simulink model "Rail_RegenerativeBraking_TianjinMetro_MotorSelection_v1"  (R2025a)
settings: Solver=ode23tb  StartTime=0.0  StopTime=SCv1.scenario.stop_time  FixedStep=Ts  MaxStep=Ts  RelTol=1e-4  EnableMultiTasking=on
PreLoadFcn:
  | SCv1_root=fileparts(fileparts(get_param(bdroot,'FileName'))); run(fullfile(SCv1_root,'config','SC_v1_parameters.m')); clear SCv1_root;
model workspace (MAT data in the model file):
  MotorCandidateIDs : object (value not decoded)
  MotorSurrogateStatement = 'parameterized surrogate traction motor model based on published nameplate data'
  TianjinMetroBaseline : object (value not decoded)
undefined symbols (not defined in the file): DiscIntNeverNeededParam, flux, Ld, Lq, Pn, SCv1, Ts
libraries: spsSeriesRLCBranchLib x5, spsControlledCurrentSourceLib x3, spsCurrentMeasurementLib x3, spsVoltageMeasurementLib x3, powerlib_extras x2, spsDCVoltageSourceLib x1, spsDiodeLib x1, spsPermanentMagnetSynchronousMachineLib x1, simulink x1, spsUniversalBridgeLib x1, sps_lib x1
(part 2 of 2)

== matlab function Rail_RegenerativeBraking_TianjinMetro_MotorSelection_v1/VehicleDynamics/Longitudinal_Dynamics ==
  data: omega_m input; v_train output; Te input; Fmechanical input; grade input; mu input; mass input; wheel_radius input; gear_ratio input; gear_efficiency input; drive_units input; A input; B input; C input; g input; Fmotor output; Fresistance output; Fadhesion_max output; Tload output
function [v_train,Fmotor,Fresistance,Fadhesion_max,Tload] = fcn(omega_m,Te,Fmechanical,grade,mu,mass,wheel_radius,gear_ratio,gear_efficiency,drive_units,A,B,C,g)
v_signed = omega_m * wheel_radius / gear_ratio;
v_train = max(v_signed,0);
Fmotor = drive_units * Te * gear_ratio * gear_efficiency / wheel_radius;
Fadhesion_max = max(mu,0) * max(mass,1) * g;
dirMotion = sign(v_signed);
if abs(v_signed) < 0.05
    dirMotion = sign(Te);
end
if dirMotion == 0
    dirMotion = 1;
end
Fdavis = A + B*abs(v_signed) + C*v_signed*v_signed;
if abs(v_signed) < 0.02 && abs(Te) < 1
    Fdavis = 0;
end
Fgrade = mass*g*grade;
Fresistance = dirMotion*Fdavis + Fgrade;
FmechLimited = min(max(Fmechanical,0),Fadhesion_max);
Fload = Fresistance + dirMotion*FmechLimited;
Tload = (Fload/drive_units)*wheel_radius/(gear_ratio*gear_efficiency);
end

== matlab function Rail_RegenerativeBraking_TianjinMetro_MotorSelection_v1/TractionBrakeSupervisor/Brake_Blend_Logic ==
  data: Traw input; Tmotor_ref output; v_train input; BrakeCmd input; SOCsc input; Udc input; mu input; mass input; SC_Enable input; Usc input; torque_limit input; drive_units input; gear_ratio input; gear_efficiency input; wheel_radius input; g input; decel input; v_zero input; v_full input; Udc_reduce input; Udc_max input; SOCmax input; Iscmax input; Umin input; PnoSC input; Fmechanical_ref output; Fregen output; BrakeActive output
function [Tmotor_ref,Fmechanical_ref,Fregen,BrakeActive] = fcn(Traw,v_train,BrakeCmd,SOCsc,Udc,mu,mass,SC_Enable,Usc,torque_limit,drive_units,gear_ratio,gear_efficiency,wheel_radius,g,decel,v_zero,v_full,Udc_reduce,Udc_max,SOCmax,Iscmax,Umin,PnoSC)

Fadh = max(mu,0)*max(mass,1)*g;
Tadh = Fadh*wheel_radius/(max(drive_units,1)*gear_ratio*gear_efficiency);
if BrakeCmd > 0.5
    BrakeActive = 1;
    Freq = min(mass*decel,Fadh);
    if v_train <= v_zero
        flow = 0;
    elseif v_train >= v_full
        flow = 1;
    else
        flow = (v_train-v_zero)/(v_full-v_zero);
    end
    fdc = min(max((Udc_max-Udc)/max(Udc_max-Udc_reduce,1),0),1);
    fsc = min(max((SOCmax-SOCsc)/0.02,0),1);
    if SC_Enable > 0.5
        Pcap = Iscmax*max(Usc,Umin)*fsc;
    else
        Pcap = PnoSC;
    end
    omega = max(v_train*gear_ratio/wheel_radius,20);
    Tpower = Pcap/(max(drive_units,1)*omega);
    Tneed = Freq*wheel_radius/(max(drive_units,1)*gear_ratio*gear_efficiency);
    Tregen = min([torque_limit,Tadh,Tpower,Tneed])*flow*fdc;
    Tregen = max(Tregen,0);
    Tmotor_ref = -Tregen;
    Fregen = drive_units*Tregen*gear_ratio*gear_efficiency/wheel_radius;
    Fmechanical_ref = max(Freq-Fregen,0);
else
    BrakeActive = 0;
    Tmotor_ref = min(max(Traw,0),min(torque_limit,Tadh));
    Fregen = 0;
    Fmechanical_ref = 0;
end
end
